simulink model "danxiangquanbozhengliudianlu_R"  (R2025a)
settings: Solver=VariableStepAuto  StartTime=0.0  StopTime=0.2  RelTol=1e-3
libraries: spsMultimeterLib x2, spsThyristorLib x2, spsACVoltageSourceLib x1, spsLinearTransformerLib x1, spsSeriesRLCBranchLib x1, sps_lib x1
settings Model: Creator=小鱼  LastModifiedBy=小鱼

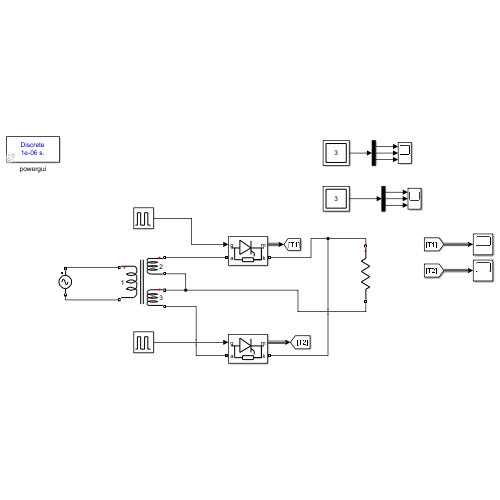
[thumbnail: Simulink's stored preview of the top-level diagram]
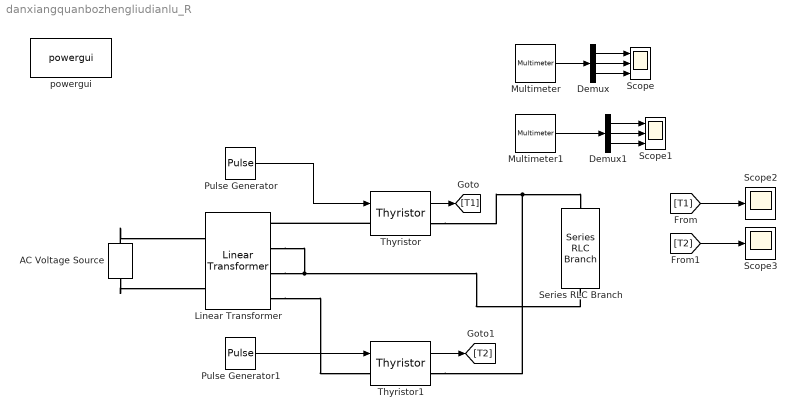
== system danxiangquanbozhengliudianlu_R ==
  AC Voltage Source : spsACVoltageSourceLib/AC Voltage Source  Amplitude=220*sqrt(2)  Phase=0  Frequency=50  SampleTime=-1  Measurements=Voltage  BusType=swing  Pref=10e3  Qref=0  Qmin=-inf  Qmax=+inf
  Demux : Demux  Outputs=3
  Demux1 : Demux  Outputs=3
  Linear Transformer : spsLinearTransformerLib/Linear Transformer  UNITS=pu  NominalPower=[ 10000 50 ]  winding1="[ 220  0 0 ]"  winding2="[ 220  0  0 ]"  ThreeWindings=on  winding3=[ 220 0 0 ]  RmLm=[ 500 500 ]  Measurements=All voltages and currents  DataType=off
  Multimeter : spsMultimeterLib/Multimeter  L=12  sel=[5 1 6]  yselected={}  Gain=[1 1 1]  OutputType=Complex  PlotAtSimulationStop=off  PhasorSimulation=off
  Multimeter1 : spsMultimeterLib/Multimeter  L=12  sel=[7 8 9]  yselected={}  Gain=[1 1 1]  OutputType=Complex  PlotAtSimulationStop=off  PhasorSimulation=off
  Pulse Generator : DiscretePulseGenerator  PulseType=Time based  Period=0.02  PulseWidth=5  PhaseDelay=60/360*0.02
  Pulse Generator1 : DiscretePulseGenerator  PulseType=Time based  Period=0.02  PulseWidth=5  PhaseDelay=(180+60)/360*0.02
  Scope : Scope  NumInputPorts=3
      settings: ActiveDisplayYMinimum=-388.90872965574863  ActiveDisplayYMaximum=388.90872965561863
  Scope1 : Scope  NumInputPorts=3
      settings: ActiveDisplayYMinimum=-38.952511712567791  ActiveDisplayYMaximum=38.952511710481879
  Scope2 : Scope
      settings: ActiveDisplayYMinimum=-732.78535879178924  ActiveDisplayYMaximum=380.83886979768386  DataLoggingVariableName=ScopeData2
  Scope3 : Scope
      settings: ActiveDisplayYMinimum=-732.78535879166657  ActiveDisplayYMaximum=380.83886979739151  DataLoggingVariableName=ScopeData3
  Series RLC Branch : spsSeriesRLCBranchLib/Series RLC Branch  LConnTagsString=__new0  RConnTagsString=__new0  BranchType=R  Resistance=10  Inductance=1e-3  SetiL0=off  InitialCurrent=0  Capacitance=1e-6  Setx0=off  InitialVoltage=0  Measurements=Branch voltage and current
  Thyristor : spsThyristorLib/Thyristor  Ron=0.001  Lon=0  Vf=0.8  IC=0  Rs=500  Cs=250e-9  Measurements=on
  Thyristor1 : spsThyristorLib/Thyristor  Ron=0.001  Lon=0  Vf=0.8  IC=0  Rs=500  Cs=250e-9  Measurements=on
  powergui : sps_lib/powergui  Priority=1  SimulationMode=Discrete  SampleTime=1e-6  frequency=60  Iterations=50  frequencyindice=50  Pbase=100e6  ErrMax=1e-4  UnitsV=kV  UnitsW=MW  buscounter=0  FunctionMessages=off  echomessages=off  EnableUseOfTLC=off  CurrentSourceSwitches=off  DisableSnubberDevices=off  DisableRonSwitches=off  DisableVfSwitches=off  DisplayEquations=off  AutomaticDiscreteSolvers=off  SolverType=Tustin/Backward Euler (TBE)  Interpol=off  ExternalGateDelay=off  methode=off  Ts=100  x0status=blocks  SPID=on  SwTol=0  HookPort=off  NonlinearTolerance=1e-4  nMaxIteration=100  ContinueOnMaxIteration=off  RestoreLinks=warning  ResistiveCurrentMeasurement=off  Frange=[0:2:500]  Ylog=off  Xlog=on  ShowGrid=off  save=off  variable=ZData  structure=0  ZoomFFT=off  StartTime=0.0  cycles=1  DisplayStyle=1  fundamental=60  FreqAxis=off  MaxFrequency=1000  frequencyindicesteady=1  RmsSteady=1  display=off
  wires:
  Pulse Generator/1 -> Thyristor/1
  Pulse Generator1/1 -> Thyristor1/1
  Multimeter/1 -> Demux/1
  Demux/1 -> Scope/1
  Demux/2 -> Scope/2
  Demux/3 -> Scope/3
  Demux1/1 -> Scope1/1
  Demux1/3 -> Scope1/3
  Demux1/2 -> Scope1/2
  Multimeter1/1 -> Demux1/1
  Thyristor1/1 -> [T2]
  Thyristor/1 -> [T1]
  [T1] -> Scope2/1
  [T2] -> Scope3/1
  connections:
  AC Voltage Source/RConn1 -- Linear Transformer/LConn1
  AC Voltage Source/LConn1 -- Linear Transformer/LConn2
  Thyristor/LConn1 -- Linear Transformer/RConn1
  Linear Transformer/RConn4 -- Thyristor1/LConn1
  Thyristor/RConn1 -- Thyristor1/RConn1 -- Series RLC Branch/LConn1
  Linear Transformer/RConn3 -- Linear Transformer/RConn2 -- Series RLC Branch/RConn1
